simulink model "LOS_Tracking"  (R2021b)
settings: Solver=VariableStepAuto  StartTime=0.0  StopTime=273.72  RelTol=1e-3
values from neighbouring files (symbols this model uses):
  EL = out.EL    [plot_result.m]
undefined symbols (not defined in the file or in its folder): AZ, Optics
libraries: slpidlib x10, simulink_extras x10
(part 2 of 2)

== matlab function LOS_Tracking/Longitudinal Velocity of Camera ==
  data: Vx input; lon_Vel_Cam output; Vy input; Vz input; p input; q input; r input; psi_AZ input; theta_EL input
function lon_Vel_Cam  = longitudinal_Velocity_Camera(Vx, Vy, Vz, p, q, r, psi_AZ, theta_EL)
    % =====================================================================
    % HÀM XÁC ĐỊNH VẬN TỐC DÀI CỦA CAMERA TRONG HỆ CAMERA
    % Phục vụ tính toán Ma trận tương tác IBVS
    % 
    % Đầu vào (Từ cảm biến UAV hoặc tín hiệu giả lập):
    %   - v_b: Vận tốc dài của UAV trong hệ Body [Vx; Vy; Vz] (m/s)
    %   - omega_b: Vận tốc góc của UAV trong hệ Body [p; q; r] (rad/s)
    %   - r_c: Vector vị trí gắn camera so với trọng tâm UAV (m)
    %   - theta_AZ, theta_EL: Góc Gimbal hiện tại phản hồi về (rad)
    % 
    % Đầu ra:
    %   - lon_Vel_Cam: Vận tốc dài của camera 
    % =====================================================================
    

    % Vận tốc dài của UAV trong hệ body
    v_b = [Vx; Vy; Vz];
    % Vận tốc góc của UAV trong hệ body
    omega_b = [p; q; r];
    % Camera được gắn ở trọng tâm
    r_c = [0; 0; 0];

    % 1. TÍNH VẬN TỐC TỊNH TIẾN TẠI ĐIỂM GẮN CAMERA (TRONG HỆ BODY)
    % Bao gồm vận tốc bay của UAV cộng với vận tốc văng do UAV bị lắc
    v_camera_body = v_b + cross(omega_b, r_c);

    % 2. MA TRẬN CHUYỂN ĐỔI: HỆ BODY -> HỆ GIMBAL NGOÀI (AZIMUTH)
    R_Body_to_AZ = [
        cos(psi_AZ),  sin(psi_AZ), 0;
       -sin(psi_AZ),  cos(psi_AZ), 0;
        0,              0,             1
    ];

    % 3. MA TRẬN CHUYỂN ĐỔI: HỆ AZIMUTH -> HỆ CAMERA (ELEVATION)
    R_AZ_to_Cam = [
        cos(theta_EL), 0, -sin(theta_EL);
        0,             1,  0;
        sin(theta_EL), 0,  cos(theta_EL)
    ];

    % 4. XUẤT RA VẬN TỐC TRONG HỆ CAMERA
    lon_Vel_Cam = R_AZ_to_Cam * R_Body_to_AZ * v_camera_body;

end

== matlab function LOS_Tracking/Gimbal ==
  data: T_AZ input; omegaAe_dot output; T_EL input; TfAz input; TfEl input; omegaAr input; omegaAe input; omegaAd input; omegaBn input; omegaBn_dot input; omegaBe input; omegaBk input; AZ input; EL input; epsilon input; epsilon_dot input; omegaBk_dot output
function [omegaAe_dot, omegaBk_dot] = Gimbal(T_AZ, T_EL, TfAz, TfEl, omegaAr, omegaAe, omegaAd, omegaBn, omegaBn_dot, omegaBe, omegaBk, AZ, EL, epsilon, epsilon_dot)
EL_Jx = EL(1);
EL_Jy = EL(2);
EL_Jz = EL(3);
AZ_Jx = AZ(1);
AZ_Jy = AZ(2);
AZ_Jz = AZ(3);

%% Phương trình động lực học cho khớp quay thứ 2
Tdel = (EL_Jz - EL_Jx) * omegaAr * omegaAd;
omegaAe_dot = (T_EL + TfEl + Tdel)/EL_Jy;

%% Phương trình động lực học cho khớp quay thứ 1
Jeq = AZ_Jz + EL_Jx * sin(epsilon)^2 + EL_Jz * cos(epsilon)^2;
Td1 = (AZ_Jx + EL_Jx * cos(epsilon)^2 + EL_Jz * sin(epsilon)^2 - AZ_Jy - EL_Jy) * omegaBn * omegaBe;
Td2 = -(EL_Jz - EL_Jx) * sin(epsilon) * cos(epsilon) * (omegaBn_dot - omegaBe * omegaBk);
Td3 = epsilon_dot * (EL_Jx - EL_Jz) * (omegaBn * cos(2*epsilon) - omegaBk*sin(2*epsilon)) + epsilon_dot * ((omegaAe + omegaBe) - EL_Jy * omegaBn);
omegaBk_dot = (T_AZ + TfAz + Td1 + Td2 + Td3)/Jeq;
end

== matlab function LOS_Tracking/Kinematic ==
  data: eta input; omegaBn output; omegaBk input; epsilon input; omegaAe input; roll input; pitch input; yaw input; omegaBe output; omegaAr output; omegaAd output; eta_dot output; epsilon_dot output
function [omegaBn, omegaBe, omegaAr, omegaAd, eta_dot, epsilon_dot] = Kinematic(eta, omegaBk, epsilon, omegaAe, roll, pitch, yaw)
%% Trục ngoài
omegaBn = roll * cos(eta) + pitch * sin(eta);
omegaBe = -roll * sin(eta) + pitch * cos(eta);
eta_dot = omegaBk - yaw;

%% Trục trong
omegaAr = omegaBn * cos(epsilon) - omegaBk * sin(epsilon);
epsilon_dot = omegaAe - omegaBe;
omegaAd = omegaBn * sin(epsilon) + omegaBk * cos(epsilon);
end
